simulink model "heli_q8_lab3_2020b"  (R2020b)
settings: Solver=ode1  StartTime=0.0  StopTime=inf  FixedStep=0.002  RelTol=1e-3  EnableMultiTasking=on
PostLoadFcn:
  | qc_set_target_type(getConfigSet(bdroot, 'QUARC Default Target Configuration'));
values from neighbouring files (symbols this model uses):
  A_est = [0 1 0 0 0 ... (first row only)    [init_heli_3_10_part_4.m]
  B_est = [0  0 ... (first row only)    [init_heli_3_10_part_4.m]
  C_est = eye(5)    [init_heli_3_10_part_4.m]
  elev_const = 0.53    [init_heli_3_10_part_4.m]
  F_2 = [K_2(1,1) K_2(1,3) ... (first row only)    [init_heli_3_10_part_4.m]
  gyro_bias = [0.0392850152533 -0.00867648252983 0.000660862987064]    [imu_bias.mat]    (also in update_imu_bias.m = mean(d(idx,13:15))')
  imu_bias = [-0.0918732538603 0 0.0496947738021 0 0]    [imu_bias.mat]    (also in update_imu_bias.m = imu_bias + mean(d(idx,2:6) - d(idx,8:12))')
  Joystick_gain_x = 1    [init_heli_3_10_part_4.m]
  Joystick_gain_y = -1    [init_heli_3_10_part_4.m]
  K_2 = lqr(A_lqr,B_lqr,Q_lqr, R_lqr)    [init_heli_3_10_part_4.m]
  L_est = transpose(place(transpose(A_est),transpose(C_est),p_est))    [init_heli_3_10_part_4.m]
  V_s_0 = 7.77    [init_heli_3_10_part_4.m]
undefined symbols (not defined in the file or in its folder): HIL, qc_get_step_size, sigbuilder_block
libraries: quarc_library x9
settings Model: SimulationMode=external  ExtModeTrigDuration=50000  Creator=Rchan  LastModifiedBy=saavim
settings SolverCC: PositivePriorityOrder=on
settings DataIOCC: LimitDataPoints=on  SaveFormat=Array  SignalLoggingSaveFormat=ModelDataLogs  ReturnWorkspaceOutputs=off
settings OptimizationCC: ExpressionDepthLimit=2147483647  InitFltsAndDblsToZero=on  LifeSpan=inf
settings DebuggingCC: SaveWithParameterizedLinksMsg=none  UnderspecifiedInitializationDetection=Classic  MergeDetectMultiDrivingBlocksExec=none  SolverPrmCheckMsg=warning  MultiTaskDSMMsg=warning  MultiTaskCondExecSysMsg=none  FcnCallInpInsideContextMsg=warning  AllowSymbolicDim=off  StateNameClashWarn=warning  SFUnexpectedBacktrackingDiag=warning  SFNoUnconditionalDefaultTransitionDiag=warning  SFExecutionAtInitializationDiag=none  ArithmeticOperatorsInVariantConditions=warning
settings HardwareCC: ProdBitPerPointer=32  ProdBitPerSizeT=32  ProdBitPerPtrDiffT=32  ProdLargestAtomicFloat=None  ProdIntDivRoundTo=Undefined  ProdEndianess=Unspecified  ProdWordSize=32  ProdHWDeviceType=32-bit Generic
settings ModelReferenceCC: PropagateSignalLabelsOutOfModel=off
settings SFSimCC: SimUseLocalCustomCode=off  CustomCodeUndefinedFunction=UseInterfaceOnly
settings RTWCC: Description=QUARC Win64 Target  SystemTargetFile=quarc_win64.tlc  TemplateMakefile=quarc_default_tmf  RTWUseLocalCustomCode=off
settings CodeAppCC: StateflowObjectComments=on
settings STFCustomTargetCC: MatFileLogging=on
settings GRTTargetCC: TargetLangStandard=C89/C90 (ANSI)  ParMdlRefBuildCompliant=off  CompOptLevelCompliant=off  CombineOutputUpdateFcns=off  GRTInterface=on  UseToolchainInfoCompliant=off  ExtMode=on  ExtModeMexFile=quarc_comm
settings ConfigComp: CovMetricSettings=de  CovSaveCumulativeToWorkspaceVar=on  CovSaveSingleToWorkspaceVar=on  CovExternalEMLEnable=off  CovSFcnEnable=off

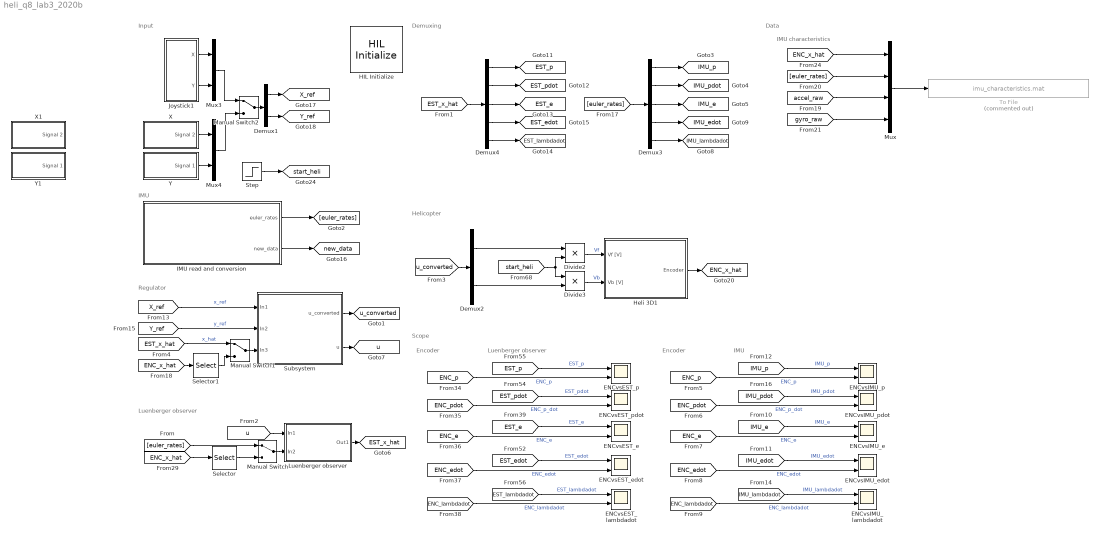
== system heli_q8_lab3_2020b ==
  note: IMU characteristics
  note: Demuxing
  note: Helicopter
  note: Luenberger observer
  note: Regulator
  note: Input
  note: IMU
  note: Scope
  note: Data
  note: Luenberger observer
  note: Encoder
  note: IMU
  note: Encoder
  Demux1 : Demux  Outputs=2
  Demux2 : Demux  Outputs=2
  Demux3 : Demux  Outputs=5
  Demux4 : Demux  Outputs=5
  Divide2 : Product  Inputs=**
  Divide3 : Product  Inputs=**
  ENCvsEST_e : Scope  NumInputPorts=2
  ENCvsEST_edot : Scope  NumInputPorts=2
  ENCvsEST_lambdadot : Scope  NumInputPorts=2
  ENCvsEST_p : Scope  NumInputPorts=2
  ENCvsEST_pdot : Scope  NumInputPorts=2
  ENCvsIMU_e : Scope  NumInputPorts=2
  ENCvsIMU_edot : Scope  NumInputPorts=2
  ENCvsIMU_lambdadot : Scope  NumInputPorts=2
  ENCvsIMU_p : Scope  NumInputPorts=2
  ENCvsIMU_pdot : Scope  NumInputPorts=2
  HIL Initialize : quarc_library/Data Acquisition/Generic/Configuration/HIL Initialize  Priority=-99  object_name=HIL-1  board_type=q8_usb  board_number=0  board_options=update_rate=normal;decimation=1  exclusive=off  active=off  hardware_clocks=[0:2]  clock_modes=[]  initial_clock_frequencies=[]  set_clock_params_at_start=off  set_clock_params_at_switch_in=off  set_clock_frequencies_at_start=off  set_clock_frequencies_at_switch_in=off  analog_input_channels=[0:7]  analog_input_configurations=[]  analog_input_maximums=10  analog_input_minimums=-10  set_analog_input_params_at_start=on  set_analog_input_params_at_switch_in=off  analog_output_channels=[0:7]  analog_output_maximums=10  analog_output_minimums=-10  initial_analog_outputs=[0]  final_analog_outputs=[0]  watchdog_analog_outputs=0  set_analog_output_params_at_start=on  set_analog_output_params_at_switch_in=off  set_analog_outputs_at_start=on  set_analog_outputs_at_switch_in=off  set_analog_outputs_at_terminate=on  set_analog_outputs_at_switch_out=off  set_analog_outputs_on_watchdog=off  digital_input_channels=[]  digital_output_channels=[]  digital_output_configuration=[]  initial_digital_outputs=[1]  final_digital_outputs=[1]  watchdog_digital_outputs=[1]  set_digital_output_params_at_start=off  set_digital_output_params_at_switch_in=off  set_digital_outputs_at_start=on  set_digital_outputs_at_switch_in=off  set_digital_outputs_at_terminate=on  set_digital_outputs_at_switch_out=off  set_digital_outputs_on_watchdog=off  encoder_channels=[0:7]  quadrature=[4]  encoder_filter_frequency=[]  initial_encoder_counts=[0]  set_encoder_params_at_start=on  set_encoder_params_at_switch_in=off  set_encoder_counts_at_start=on  set_encoder_counts_at_switch_in=off  pwm_channels=[0:7]  pwm_modes=0  pwm_frequency=99.532799999999995e6/4095  pwm_configuration=[0]  pwm_alignment=[0]  pwm_polarity=[1]  pwm_leading_deadband=[0]  pwm_trailing_deadband=[0]  initial_pwm_outputs=[0]  final_pwm_outputs=[0]  watchdog_pwm_outputs=[0]  set_pwm_params_at_start=on  set_pwm_params_at_switch_in=off  set_pwm_outputs_at_start=on  set_pwm_outputs_at_switch_in=off  set_pwm_outputs_at_terminate=on  set_pwm_outputs_at_switch_out=off  set_pwm_outputs_on_watchdog=off  other_output_channels=[]  initial_other_outputs=[]  final_other_outputs=[]  watchdog_other_outputs=[]  set_other_outputs_at_start=off  set_other_outputs_at_switch_in=off  set_other_outputs_at_terminate=off  set_other_outputs_at_switch_out=off  set_other_outputs_on_watchdog=off
  Heli 3D1 : Subsystem
  IMU read and conversion : Subsystem
  Joystick1 : Subsystem
  Luenberger observer : Subsystem
  Manual Switch : ManualSwitch
  Manual Switch1 : ManualSwitch
  Manual Switch2 : ManualSwitch
  Mux : Mux
  Mux3 : Mux  Inputs=2
  Mux4 : Mux  Inputs=2
  Selector : Selector  InputPortWidth=6  IndexOptions=Index vector (dialog)  Indices=[1 2 3 4 6]  OutputSizes=1
  Selector1 : Selector  InputPortWidth=6  IndexOptions=Index vector (dialog)  Indices=[1 2 3 4 6]  OutputSizes=1
  Step : Step  Time=3  SampleTime=0
  Subsystem : Subsystem
  To File : ToFile  Commented=on  Filename=imu_characteristics.mat  MatrixName=imu_characteristics  SampleTime=0.002
  X : Subsystem  Tag=STV Subsys  LoadFcn=sigbuilder_block('load');  StartFcn=sigbuilder_block('start');  StopFcn=sigbuilder_block('stop');  ClipboardFcn=sigbuilder_block('clipboard');  mask(Sigbuilder block){tuvar=[0:10]}
      mask help: Simulink:masks:SigbuilderBlock_MD
      mask init:
      | if ~strcmp(get_param(bdroot(gcbh),'SimulationStatus'),'stopped') tuvar = sigbuilder_block('maskInit'); end
      settings: CopyFcn=sigbuilder_block('copy');  DeleteFcn=sigbuilder_block('delete');  ModelCloseFcn=sigbuilder_block('modelClose');  PreSaveFcn=sigbuilder_block('preSave');  PauseFcn=sigbuilder_block('pause');  ContinueFcn=sigbuilder_block('continue');  NameChangeFcn=sigbuilder_block('namechange');  OpenFcn=sigbuilder_block('open',[0 172 1440 619 ]);  CloseFcn=sigbuilder_block('close');
      mask Display: plot(0, 0, 100, 100,[2, 2, 32, 32, 2], [68, 8, 8, 68, 68],[32, 2], [38, 38], [32, 19, 2],[53, 60, 44], [32, 17, 17, 2],[16, 16, 31, 31]);txt = getActiveGroup(gcbh);text(2, 100, txt,'verticalAlignment', 'top');
  X1 : Subsystem  Tag=STV Subsys  LoadFcn=sigbuilder_block('load');  StartFcn=sigbuilder_block('start');  StopFcn=sigbuilder_block('stop');  ClipboardFcn=sigbuilder_block('clipboard');  mask(Sigbuilder block){tuvar=[0:10]}
      mask help: Simulink:masks:SigbuilderBlock_MD
      mask init:
      | if ~strcmp(get_param(bdroot(gcbh),'SimulationStatus'),'stopped') tuvar = sigbuilder_block('maskInit'); end
      settings: CopyFcn=sigbuilder_block('copy');  DeleteFcn=sigbuilder_block('delete');  ModelCloseFcn=sigbuilder_block('modelClose');  PreSaveFcn=sigbuilder_block('preSave');  PauseFcn=sigbuilder_block('pause');  ContinueFcn=sigbuilder_block('continue');  NameChangeFcn=sigbuilder_block('namechange');  OpenFcn=sigbuilder_block('open',[0 172 1440 619 ]);  CloseFcn=sigbuilder_block('close');
      mask Display: plot(0, 0, 100, 100,[2, 2, 32, 32, 2], [68, 8, 8, 68, 68],[32, 2], [38, 38], [32, 19, 2],[53, 60, 44], [32, 17, 17, 2],[16, 16, 31, 31]);txt = getActiveGroup(gcbh);text(2, 100, txt,'verticalAlignment', 'top');
  Y : Subsystem  Tag=STV Subsys  LoadFcn=sigbuilder_block('load');  StartFcn=sigbuilder_block('start');  StopFcn=sigbuilder_block('stop');  ClipboardFcn=sigbuilder_block('clipboard');  mask(Sigbuilder block){tuvar=[0:10]}
      mask help: Simulink:masks:SigbuilderBlock_MD
      mask init:
      | if ~strcmp(get_param(bdroot(gcbh),'SimulationStatus'),'stopped') tuvar = sigbuilder_block('maskInit'); end
      settings: CopyFcn=sigbuilder_block('copy');  DeleteFcn=sigbuilder_block('delete');  ModelCloseFcn=sigbuilder_block('modelClose');  PreSaveFcn=sigbuilder_block('preSave');  PauseFcn=sigbuilder_block('pause');  ContinueFcn=sigbuilder_block('continue');  NameChangeFcn=sigbuilder_block('namechange');  OpenFcn=sigbuilder_block('open',[217.5 306 1336.5 574.5 ]);  CloseFcn=sigbuilder_block('close');
      mask Display: plot(0, 0, 100, 100,[2, 2, 32, 32, 2], [68, 8, 8, 68, 68],[32, 2], [38, 38], [32, 19, 2],[53, 60, 44], [32, 17, 17, 2],[16, 16, 31, 31]);txt = getActiveGroup(gcbh);text(2, 100, txt,'verticalAlignment', 'top');
  Y1 : Subsystem  Tag=STV Subsys  LoadFcn=sigbuilder_block('load');  StartFcn=sigbuilder_block('start');  StopFcn=sigbuilder_block('stop');  ClipboardFcn=sigbuilder_block('clipboard');  mask(Sigbuilder block){tuvar=[0:10]}
      mask help: Simulink:masks:SigbuilderBlock_MD
      mask init:
      | if ~strcmp(get_param(bdroot(gcbh),'SimulationStatus'),'stopped') tuvar = sigbuilder_block('maskInit'); end
      settings: CopyFcn=sigbuilder_block('copy');  DeleteFcn=sigbuilder_block('delete');  ModelCloseFcn=sigbuilder_block('modelClose');  PreSaveFcn=sigbuilder_block('preSave');  PauseFcn=sigbuilder_block('pause');  ContinueFcn=sigbuilder_block('continue');  NameChangeFcn=sigbuilder_block('namechange');  OpenFcn=sigbuilder_block('open',[217.5 306 1336.5 574.5 ]);  CloseFcn=sigbuilder_block('close');
      mask Display: plot(0, 0, 100, 100,[2, 2, 32, 32, 2], [68, 8, 8, 68, 68],[32, 2], [38, 38], [32, 19, 2],[53, 60, 44], [32, 17, 17, 2],[16, 16, 31, 31]);txt = getActiveGroup(gcbh);text(2, 100, txt,'verticalAlignment', 'top');
  tag scope: ENC_x_hat=global, EST_e=global, EST_edot=global, EST_lambdadot=global, EST_p=global, EST_pdot=global, EST_x_hat=global, IMU_e=global, IMU_edot=global, IMU_lambdadot=global, IMU_p=global, IMU_pdot=global, X_ref=global, Y_ref=global, new_data=global, start_heli=global, u=global, u_converted=global
  wires:
  Demux4/1 -> [EST_p]
  Demux4/2 -> [EST_pdot]
  Demux4/3 -> [EST_e]
  Demux4/4 -> [EST_edot]
  Demux4/5 -> [EST_lambdadot]
  X/1(Signal 2) -> Mux4/1
  Manual Switch2/1 -> Demux1/1
  Y/1(Signal 1) -> Mux4/2
  Demux1/1 -> [X_ref]
  Joystick1/1(X) -> Mux3/1
  Mux3/1 -> Manual Switch2/1
  Demux1/2 -> [Y_ref]
  Joystick1/2(Y) -> Mux3/2
  Step/1 -> [start_heli]
  Mux4/1 -> Manual Switch2/2
  [EST_x_hat] -> Demux4/1
  [X_ref] -> Subsystem/1(In1)  "x_ref"
  [Y_ref] -> Subsystem/2(In2)  "y_ref"
  Subsystem/1(u_converted) -> [u_converted]
  Subsystem/2(u) -> [u]
  Manual Switch/1 -> Luenberger observer/2(In2)
  [u] -> Luenberger observer/1(In1)
  [euler_rates] -> Manual Switch/1
  Luenberger observer/1(Out1) -> [EST_x_hat]
  Demux2/1 -> Divide2/1
  Demux2/2 -> Divide3/2
  [u_converted] -> Demux2/1
  [start_heli] -> Divide3/1, Divide2/2
  Heli 3D1/1(Encoder) -> [ENC_x_hat]
  IMU read and conversion/1(euler_rates) -> [euler_rates]
  IMU read and conversion/2(new_data) -> [new_data]
  [ENC_x_hat] -> Selector/1
  Selector/1 -> Manual Switch/2
  [ENC_edot] -> ENCvsEST_edot/2  "ENC_edot"
  [ENC_lambdadot] -> ENCvsEST_lambdadot/2  "ENC_lambdadot"
  [EST_lambdadot] -> ENCvsEST_lambdadot/1  "EST_lambdadot"
  [EST_edot] -> ENCvsEST_edot/1  "EST_edot"
  [EST_p] -> ENCvsEST_p/1  "EST_p"
  [IMU_pdot] -> ENCvsIMU_pdot/1  "IMU_pdot"
  [ENC_pdot] -> ENCvsEST_pdot/2  "ENC_p_dot"
  [EST_e] -> ENCvsEST_e/1  "EST_e"
  [IMU_p] -> ENCvsIMU_p/1  "IMU_p"
  [ENC_p] -> ENCvsEST_p/2  "ENC_p"
  [ENC_edot] -> ENCvsIMU_edot/2  "ENC_edot"
  [IMU_edot] -> ENCvsIMU_edot/1  "IMU_edot"
  [ENC_lambdadot] -> ENCvsIMU_lambdadot/2  "ENC_lambdadot"
  [ENC_e] -> ENCvsEST_e/2  "ENC_e"
  [IMU_lambdadot] -> ENCvsIMU_lambdadot/1  "IMU_lambdadot"
  [EST_pdot] -> ENCvsEST_pdot/1  "EST_pdot"
  [ENC_e] -> ENCvsIMU_e/2  "ENC_e"
  [ENC_pdot] -> ENCvsIMU_pdot/2  "ENC_p_dot"
  [IMU_e] -> ENCvsIMU_e/1  "IMU_e"
  [ENC_p] -> ENCvsIMU_p/2  "ENC_p"
  [euler_rates] -> Demux3/1
  Demux3/3 -> [IMU_e]
  Demux3/4 -> [IMU_edot]
  Demux3/5 -> [IMU_lambdadot]
  Demux3/2 -> [IMU_pdot]
  Demux3/1 -> [IMU_p]
  [EST_x_hat] -> Manual Switch1/1  "x_hat"
  Manual Switch1/1 -> Subsystem/3(In3)
  Selector1/1 -> Manual Switch1/2
  [ENC_x_hat] -> Selector1/1
  [ENC_x_hat] -> Mux/1
  [euler_rates] -> Mux/2
  [accel_raw] -> Mux/3
  [gyro_raw] -> Mux/4
  Mux/1 -> To File/1
  Divide2/1 -> Heli 3D1/1(Vf [V])  "Vf"
  Divide3/1 -> Heli 3D1/2(Vb [V])  "Vb"

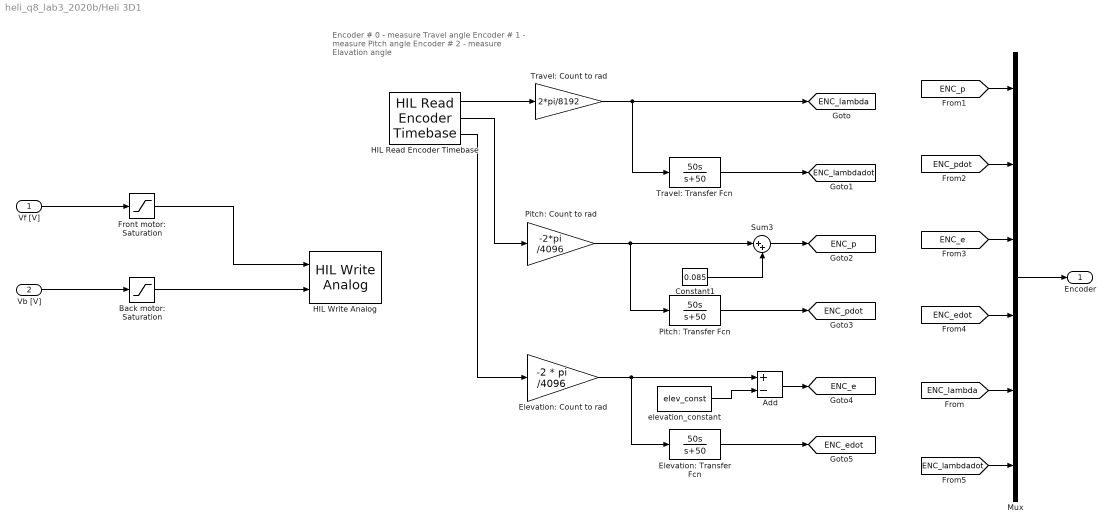
== system heli_q8_lab3_2020b/Heli 3D1 ==
  note: Encoder # 0 - measure Travel angle
      | Encoder # 1 - measure Pitch angle
      | Encoder # 2 - measure Elavation angle
  Vf [V] : Inport
  Vb [V] : Inport  Port=2
  Add : Sum  Inputs=+-
  Back motor: Saturation : Saturate  UpperLimit=5  LowerLimit=-5
  Constant1 : Constant  Value=0.085
  Elevation: Count to rad : Gain  Gain=-2 * pi /4096
  Elevation: Transfer Fcn : TransferFcn  Numerator=[50 0]  Denominator=[1 50]
  Front motor: Saturation : Saturate  UpperLimit=5  LowerLimit=-5
  HIL Read Encoder Timebase : quarc_library/Data Acquisition/Generic/Timebases/HIL Read Encoder Timebase  object_name=HIL-1  clock=0  channels=[0:2]  active=on  vector_output=off  data_type_mode=Inherit via back propagation  data_type=double  overflow_mode=Error on overflow  samples_in_buffer=max(ceil(1/qc_get_step_size), 1)
  HIL Write Analog : quarc_library/Data Acquisition/Generic/Immediate I//O/HIL Write Analog  object_name=HIL-1  channels=[0:1]  sample_time=-1  active=off  vector_input=off
  Mux : Mux  Inputs=6
  Pitch: Count to rad : Gain  Gain=-2*pi /4096
  Pitch: Transfer Fcn : TransferFcn  Numerator=[50 0]  Denominator=[1 50]
  Sum3 : Sum  Inputs=|++
  Travel: Count to rad : Gain  Gain=2*pi/8192
  Travel: Transfer Fcn : TransferFcn  Numerator=[50 0]  Denominator=[1 50]
  elevation_constant : Constant  Value=elev_const
  Encoder : Outport
  tag scope: ENC_e=global, ENC_edot=global, ENC_lambda=global, ENC_lambdadot=global, ENC_p=global, ENC_pdot=global
  wires:
  HIL Read Encoder Timebase/1 -> Travel: Count to rad/1
  HIL Read Encoder Timebase/2 -> Pitch: Count to rad/1
  HIL Read Encoder Timebase/3 -> Elevation: Count to rad/1
  Travel: Count to rad/1 -> Travel: Transfer Fcn/1, [ENC_lambda]
  Travel: Transfer Fcn/1 -> [ENC_lambdadot]
  Elevation: Count to rad/1 -> Add/1, Elevation: Transfer Fcn/1
  Elevation: Transfer Fcn/1 -> [ENC_edot]
  Vf [V]/1 -> Front motor: Saturation/1
  Vb [V]/1 -> Back motor: Saturation/1
  Front motor: Saturation/1 -> HIL Write Analog/1
  Back motor: Saturation/1 -> HIL Write Analog/2
  elevation_constant/1 -> Add/2
  Add/1 -> [ENC_e]
  Pitch: Count to rad/1 -> Pitch: Transfer Fcn/1, Sum3/1
  Pitch: Transfer Fcn/1 -> [ENC_pdot]
  Constant1/1 -> Sum3/2
  Sum3/1 -> [ENC_p]
  Mux/1 -> Encoder/1
  [ENC_p] -> Mux/1
  [ENC_pdot] -> Mux/2
  [ENC_lambdadot] -> Mux/6
  [ENC_lambda] -> Mux/5
  [ENC_edot] -> Mux/4
  [ENC_e] -> Mux/3

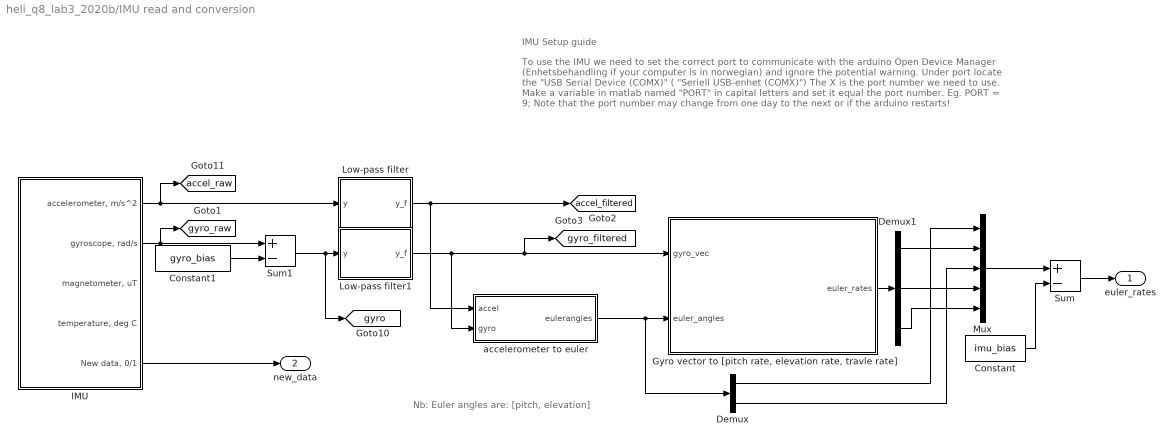
== system heli_q8_lab3_2020b/IMU read and conversion ==
  note: Nb: Euler angles are: [pitch, elevation]
  note: IMU Setup guide
  note: To use the IMU we need to set the correct port to communicate with the arduino
      | Open Device Manager (Enhetsbehandling if your computer is in norwegian) and ignore the potential warning.
      | Under port locate the "USB Serial Device (COMX)" ( "Seriell USB-enhet (COMX)")
      | The X is the port number we need to use.
      |
      | Make a variable in matlab named "PORT" in capital letters and set it equal the port number.
      | Eg.
      | PORT = 9;
      |
      | Note that the port number may change from one day to the next or if the arduino restarts!
  Constant : Constant  Value=imu_bias
  Constant1 : Constant  Value=gyro_bias
  Demux : Demux  Outputs=2
  Demux1 : Demux  Outputs=3
  "Gyro vector to [pitch rate, elevation rate, travle rate]" : MATLAB Function  TreatAsAtomicUnit=on
  IMU : Subsystem
  Low-pass filter : MATLAB Function  TreatAsAtomicUnit=on
  Low-pass filter1 : MATLAB Function  TreatAsAtomicUnit=on
  Mux : Mux  Inputs=5
  Sum : Sum  Inputs=+-
  Sum1 : Sum  Inputs=+-
  accelerometer to euler : MATLAB Function  TreatAsAtomicUnit=on
  euler_rates : Outport
  new_data : Outport  Port=2
  tag scope: accel_filtered=global, accel_raw=global, gyro=global, gyro_filtered=global, gyro_raw=global
  wires:
  IMU/2("gyroscope, rad/s") -> Sum1/1, [gyro_raw]
  "Gyro vector to [pitch rate, elevation rate, travle rate]"/1(euler_rates) -> Demux1/1
  Demux/1 -> Mux/1
  Demux1/1 -> Mux/2
  Demux/2 -> Mux/3
  Demux1/2 -> Mux/4
  Demux1/3 -> Mux/5
  IMU/5("New data, 0/1") -> new_data/1
  IMU/1("accelerometer, m/s^2") -> [accel_raw], Low-pass filter/1(y)
  accelerometer to euler/1(eulerangles) -> Demux/1, "Gyro vector to [pitch rate, elevation rate, travle rate]"/2(euler_angles)
  Constant/1 -> Sum/2
  Constant1/1 -> Sum1/2
  Sum1/1 -> [gyro], Low-pass filter1/1(y)
  Sum/1 -> euler_rates/1
  Mux/1 -> Sum/1
  Low-pass filter/1(y_f) -> [accel_filtered], accelerometer to euler/1(accel)
  Low-pass filter1/1(y_f) -> [gyro_filtered], "Gyro vector to [pitch rate, elevation rate, travle rate]"/1(gyro_vec), accelerometer to euler/2(gyro)

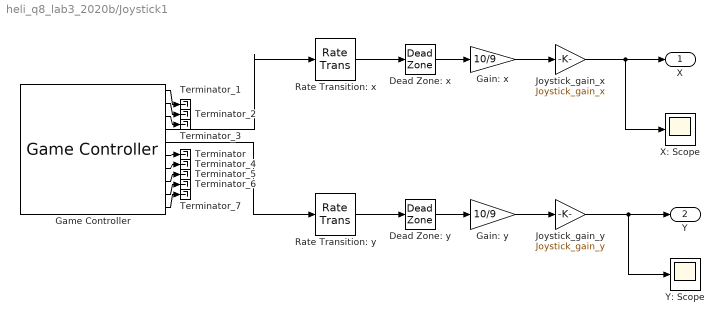
== system heli_q8_lab3_2020b/Joystick1 ==
  Dead Zone: x : DeadZone  LowerValue=-0.1  UpperValue=0.1  SaturateOnIntegerOverflow=on
  Dead Zone: y : DeadZone  LowerValue=-0.1  UpperValue=0.1  SaturateOnIntegerOverflow=on
  Gain: x : Gain  Gain=10/9
  Gain: y : Gain  Gain=10/9
  Game Controller : quarc_library/Devices/Peripherals/Target/Game Controller  controller=1  buffer_size=12  deadzone=[]  saturation=[]  sample_time=max(qc_get_step_size, 0.01)  auto_center=off  enabled=on
      settings: SourceProductName=QUARC Targets
  Joystick_gain_x : Gain  Gain=Joystick_gain_x
  Joystick_gain_y : Gain  Gain=Joystick_gain_y
  Rate Transition: x : RateTransition
  Rate Transition: y : RateTransition
  Terminator : Terminator
  Terminator_{1..7} (7 alike) : Terminator
  X: Scope : Scope
  Y: Scope : Scope
  X : Outport
  Y : Outport  Port=2
  wires:
  Rate Transition: y/1 -> Dead Zone: y/1
  Rate Transition: x/1 -> Dead Zone: x/1
  Game Controller/5 -> Rate Transition: y/1
  Game Controller/4 -> Rate Transition: x/1
  Game Controller/1 -> Terminator_1/1
  Game Controller/2 -> Terminator_2/1
  Game Controller/7 -> Terminator_4/1
  Game Controller/8 -> Terminator_5/1
  Game Controller/9 -> Terminator_6/1
  Game Controller/10 -> Terminator_7/1
  Game Controller/6 -> Terminator/1
  Dead Zone: x/1 -> Gain: x/1
  Dead Zone: y/1 -> Gain: y/1
  Gain: x/1 -> Joystick_gain_x/1
  Gain: y/1 -> Joystick_gain_y/1
  Joystick_gain_x/1 -> X/1, X: Scope/1
  Joystick_gain_y/1 -> Y: Scope/1, Y/1
  Game Controller/3 -> Terminator_3/1

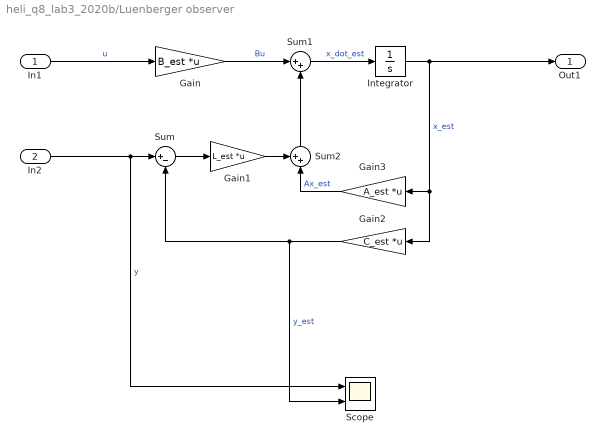
== system heli_q8_lab3_2020b/Luenberger observer ==
  In1 : Inport
  In2 : Inport  Port=2
  Gain : Gain  Gain=B_est  Multiplication=Matrix(K*u)
  Gain1 : Gain  Gain=L_est  Multiplication=Matrix(K*u)
  Gain2 : Gain  Gain=C_est  Multiplication=Matrix(K*u)
  Gain3 : Gain  Gain=A_est  Multiplication=Matrix(K*u)
  Integrator : Integrator
  Scope : Scope  NumInputPorts=2
  Sum : Sum  Inputs=|+-
  Sum1 : Sum  Inputs=|++
  Sum2 : Sum  Inputs=++|
  Out1 : Outport
  wires:
  In1/1 -> Gain/1  "u"
  In2/1 -> Scope/1, Sum/1  "y"
  Gain/1 -> Sum1/1  "Bu"
  Sum/1 -> Gain1/1
  Sum1/1 -> Integrator/1  "x_dot_est"
  Integrator/1 -> Gain2/1, Gain3/1, Out1/1  "x_est"
  Gain2/1 -> Scope/2, Sum/2  "y_est"
  Gain1/1 -> Sum2/1
  Sum2/1 -> Sum1/2
  Gain3/1 -> Sum2/2  "Ax_est"

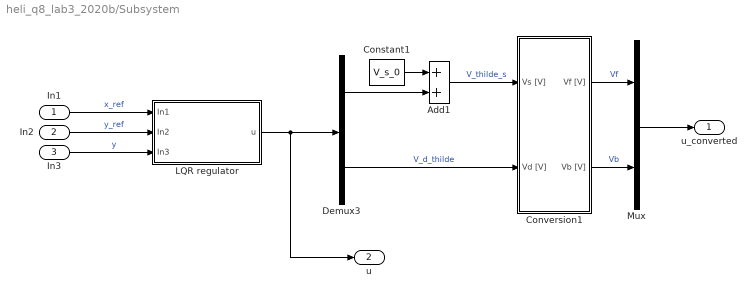
== system heli_q8_lab3_2020b/Subsystem ==
  In1 : Inport
  In2 : Inport  Port=2
  In3 : Inport  Port=3
  Add1 : Sum
  Constant1 : Constant  Value=V_s_0
  Conversion1 : Subsystem
  Demux3 : Demux  Outputs=2
  LQR regulator : Subsystem
  Mux : Mux  Inputs=2
  u_converted : Outport
  u : Outport  Port=2
  wires:
  Add1/1 -> Conversion1/1(Vs [V])  "V_thilde_s"
  Demux3/2 -> Conversion1/2(Vd [V])  "V_d_thilde"
  Conversion1/2(Vb [V]) -> Mux/2  "Vb"
  Constant1/1 -> Add1/1
  In1/1 -> LQR regulator/1(In1)  "x_ref"
  In3/1 -> LQR regulator/3(In3)  "y"
  Mux/1 -> u_converted/1
  LQR regulator/1(u) -> u/1, Demux3/1
  Conversion1/1(Vf [V]) -> Mux/1  "Vf"
  In2/1 -> LQR regulator/2(In2)  "y_ref"
  Demux3/1 -> Add1/2

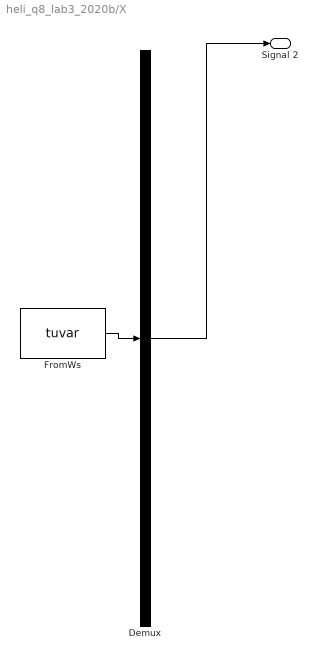
== system heli_q8_lab3_2020b/X ==
  Demux : Demux  Tag=STV Demux  Outputs=1
      settings: DisplayOption=none
  FromWs : FromWorkspace  Tag=STV FromWs  VariableName=tuvar
      SigBuilderData=|
      | common.afterFinalStr = 'Extrapolate'
      | common.sampleTime = 0
      | dataSet.timeRange = [0 90]
      | dataSet.name = 'Group 1'
      | sbobj.Groups.Name = 'Group 1'
      | sbobj.Groups.Signals.Name = 'Signal 2'
      | sbobj.Groups.Signals.XData = [0 35 35 40 40 45 45 50 50 55 55 65 65 70 70 80 80 90]
      | sbobj.Groups.Signals.YData = [0 0 0.25 0.25 0 0 -0.25 -0.25 0 0 0.099 0.099 0 0 -0.131 -0.131 0 0]
      | sbobj.Groups.TimeRange = [0 90]
  Signal 2 : Outport  Tag=STV Outport
  wires:
  Demux/1 -> Signal 2/1
  FromWs/1 -> Demux/1

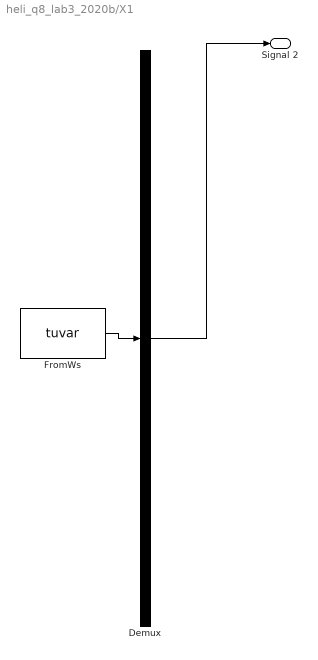
== system heli_q8_lab3_2020b/X1 ==
  Demux : Demux  Tag=STV Demux  Outputs=1
      settings: DisplayOption=none
  FromWs : FromWorkspace  Tag=STV FromWs  VariableName=tuvar
      SigBuilderData=|
      | common.afterFinalStr = 'Extrapolate'
      | common.sampleTime = 0
      | dataSet.timeRange = [0 60]
      | dataSet.name = 'Group 1'
      | sbobj.Groups.Name = 'Group 1'
      | sbobj.Groups.Signals.Name = 'Signal 2'
      | sbobj.Groups.Signals.XData = [0 10 10 15 15 30 30 35 35 60]
      | sbobj.Groups.Signals.YData = [0 0 0.4 0.4 0 0 -0.4 -0.4 0 0]
      | sbobj.Groups.TimeRange = [0 60]
  Signal 2 : Outport  Tag=STV Outport
  wires:
  Demux/1 -> Signal 2/1
  FromWs/1 -> Demux/1

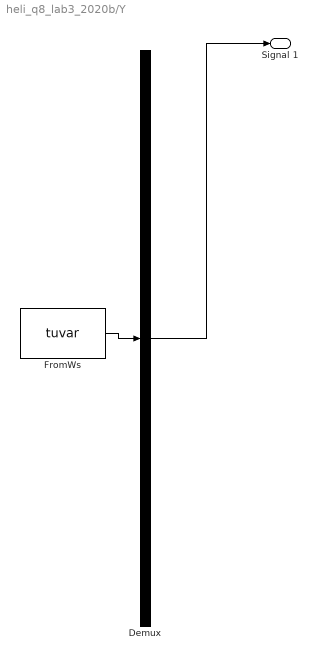
== system heli_q8_lab3_2020b/Y ==
  Demux : Demux  Tag=STV Demux  Outputs=1
      settings: DisplayOption=none
  FromWs : FromWorkspace  Tag=STV FromWs  VariableName=tuvar
      SigBuilderData=|
      | common.afterFinalStr = 'Extrapolate'
      | common.sampleTime = 0
      | dataSet.timeRange = [0 90]
      | dataSet.name = 'Group 1'
      | sbobj.Groups.Name = 'Group 1'
      | sbobj.Groups.Signals.Name = 'Signal 1'
      | sbobj.Groups.Signals.XData = [0 4 4 10 10 20 20 23 23 27 27 30 30 90]
      | sbobj.Groups.Signals.YData = [0 0 0.101 0.101 0 0 -0.2 -0.2 0 0 0.2 0.2 0 0]
      | sbobj.Groups.TimeRange = [0 90]
  Signal 1 : Outport  Tag=STV Outport
  wires:
  Demux/1 -> Signal 1/1
  FromWs/1 -> Demux/1

== system heli_q8_lab3_2020b/Y1 ==
  Demux : Demux  Tag=STV Demux  Outputs=1
      settings: DisplayOption=none
  FromWs : FromWorkspace  Tag=STV FromWs  VariableName=tuvar
      SigBuilderData=|
      | common.afterFinalStr = 'Extrapolate'
      | common.sampleTime = 0
      | dataSet.timeRange = [0 10]
      | dataSet.name = 'Group 1'
      | sbobj.Groups.Name = 'Group 1'
      | sbobj.Groups.Signals.Name = 'Signal 1'
      | sbobj.Groups.Signals.XData = [0 5.01 5.01 6 6 10]
      | sbobj.Groups.Signals.YData = [0 0 0.4 0.4 0 0]
  Signal 1 : Outport  Tag=STV Outport
  wires:
  Demux/1 -> Signal 1/1
  FromWs/1 -> Demux/1

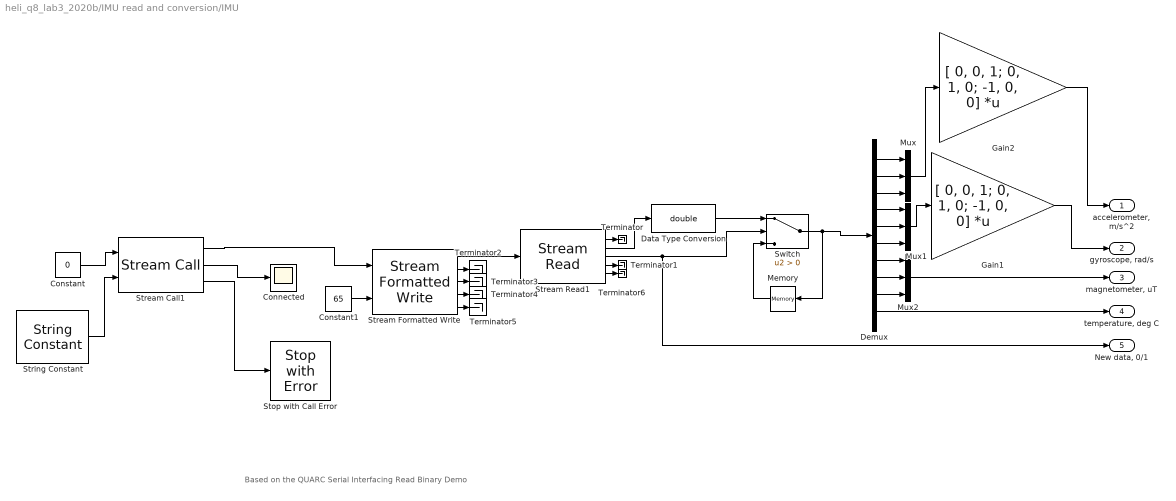
== system heli_q8_lab3_2020b/IMU read and conversion/IMU ==
  note: Based on the QUARC Serial Interfacing Read Binary Demo
  Connected : Scope
  Constant : Constant  Value=0
  Constant1 : Constant  Value=65
  Data Type Conversion : DataTypeConversion  OutDataTypeStr=double
  Demux : Demux  Outputs=10
  Gain1 : Gain  Gain=[ 0, 0, 1; 0, 1, 0; -1, 0, 0]  Multiplication=Matrix(K*u) (u vector)
  Gain2 : Gain  Gain=[ 0, 0, 1; 0, 1, 0; -1, 0, 0]  Multiplication=Matrix(K*u) (u vector)
  Memory : Memory  InitialCondition=[0 0 0 0 0 0 0 0 0 0]
  Mux : Mux  Inputs=3
  Mux1 : Mux  Inputs=3
  Mux2 : Mux  Inputs=3
  Stop with Call Error : quarc_library/Sinks/Error Handling/Stop with Error  message_type=Interpret input as error code  message=Error occurred
      settings: SourceProductName=QUARC Targets
  Stream Call1 : quarc_library/Communications/Intermediate/Stream Call  uri_source=External input port  uri=serial://IMU:9?baud=115200,word=8,parity=none,stop=1,flow='none'  apply_uri_to_all_configs=on  send_buffer_size=8000  receive_buffer_size=8000  byte_order=little endian (Intel - LSB first)  sample_time=qc_get_step_size  non_blocking=on  active=off
      settings: SourceProductName=QUARC Targets
  Stream Formatted Write : quarc_library/Communications/Intermediate/Stream Formatted Write  format_string=%c\n  max_code_units=80  optimization=Minimizing latency
      settings: SourceProductName=QUARC Targets
  Stream Read1 : quarc_library/Communications/Intermediate/Stream Read  data_type=single  type_expr=BusObject  num_elements=10  receive_dims=off
      settings: SourceProductName=QUARC Targets
  String Constant : quarc_library/Strings/String Constant  string_value=qc_perform_substitutions('serial://IMU:%{PORT}?baud=115200,word=8,parity=none,stop=1')  evaluate_string=on  string_type=URI  max_length=255  sample_time=inf  variable_size=off
      settings: AttributesFormatString="\"serial://IMU:6?baud=115200,word=8,parity=none,stop=1\""  SourceProductName=QUARC Targets
  Switch : Switch  Criteria=u2 > Threshold
  Terminator{,1..6} (7 alike) : Terminator
  "accelerometer, m/s^2" : Outport
  "gyroscope, rad/s" : Outport  Port=2
  "magnetometer, uT" : Outport  Port=3
  "temperature, deg C" : Outport  Port=4
  "New data, 0/1" : Outport  Port=5
  wires:
  Switch/1 -> Memory/1, Demux/1
  Data Type Conversion/1 -> Switch/1
  Stream Read1/3 -> "New data, 0/1"/1, Switch/2
  Stream Formatted Write/1 -> Stream Read1/1
  Constant1/1 -> Stream Formatted Write/2
  Gain1/1 -> "gyroscope, rad/s"/1
  Gain2/1 -> "accelerometer, m/s^2"/1
  Stream Read1/4 -> Terminator1/1
  Demux/10 -> "temperature, deg C"/1
  Mux1/1 -> Gain1/1
  Stream Read1/2 -> Data Type Conversion/1
  Demux/7 -> Mux2/1
  Demux/8 -> Mux2/2
  Demux/9 -> Mux2/3
  Mux2/1 -> "magnetometer, uT"/1
  Demux/6 -> Mux1/3
  Demux/5 -> Mux1/2
  Demux/4 -> Mux1/1
  Mux/1 -> Gain2/1
  Demux/3 -> Mux/3
  Demux/1 -> Mux/1
  Demux/2 -> Mux/2
  Stream Read1/1 -> Terminator/1
  Stream Call1/1 -> Stream Formatted Write/1
  Constant/1 -> Stream Call1/1
  String Constant/1 -> Stream Call1/2
  Stream Call1/2 -> Connected/1
  Stream Call1/3 -> Stop with Call Error/1
  Memory/1 -> Switch/3
  Stream Formatted Write/2 -> Terminator2/1
  Stream Formatted Write/3 -> Terminator3/1
  Stream Formatted Write/4 -> Terminator4/1
  Stream Formatted Write/5 -> Terminator5/1
  Stream Read1/5 -> Terminator6/1

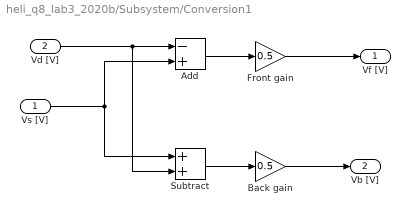
== system heli_q8_lab3_2020b/Subsystem/Conversion1 ==
  Vs [V] : Inport
  Vd [V] : Inport  Port=2
  Add : Sum  Inputs=-+
  Back gain : Gain  Gain=0.5
  Front gain : Gain  Gain=0.5
  Subtract : Sum
  Vf [V] : Outport
  Vb [V] : Outport  Port=2
  wires:
  Vd [V]/1 -> Subtract/2, Add/1
  Vs [V]/1 -> Subtract/1, Add/2
  Subtract/1 -> Back gain/1
  Back gain/1 -> Vb [V]/1
  Add/1 -> Front gain/1
  Front gain/1 -> Vf [V]/1

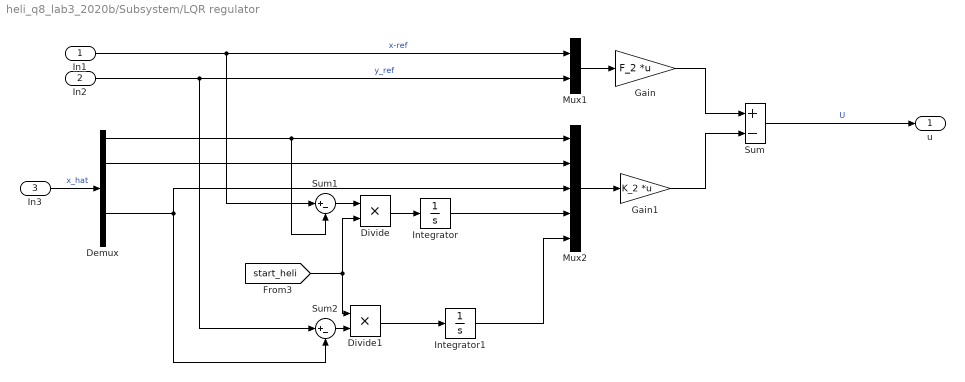
== system heli_q8_lab3_2020b/Subsystem/LQR regulator ==
  In1 : Inport
  In2 : Inport  Port=2
  In3 : Inport  Port=3
  Demux : Demux  Outputs=5
  Divide : Product  Inputs=**
  Divide1 : Product  Inputs=**
  Gain : Gain  Gain=F_2  Multiplication=Matrix(K*u)
  Gain1 : Gain  Gain=K_2  Multiplication=Matrix(K*u)
  Integrator : Integrator
  Integrator1 : Integrator
  Mux1 : Mux  Inputs=2
  Mux2 : Mux  Inputs=5
  Sum : Sum  Inputs=+-
  Sum1 : Sum  Inputs=|+-
  Sum2 : Sum  Inputs=|+-
  u : Outport
  wires:
  Demux/1 -> Sum1/2, Mux2/1
  Integrator1/1 -> Mux2/5
  Demux/2 -> Mux2/2
  Gain1/1 -> Sum/2
  Mux1/1 -> Gain/1
  Sum/1 -> u/1  "U"
  Mux2/1 -> Gain1/1
  Demux/4 -> Sum2/2, Mux2/3
  Gain/1 -> Sum/1
  Integrator/1 -> Mux2/4
  In1/1 -> Mux1/1, Sum1/1  "x-ref"
  In2/1 -> Mux1/2, Sum2/1  "y_ref"
  Sum1/1 -> Divide/1
  Divide/1 -> Integrator/1
  [start_heli] -> Divide1/1, Divide/2
  Divide1/1 -> Integrator1/1
  Sum2/1 -> Divide1/2
  In3/1 -> Demux/1  "x_hat"

== matlab function heli_q8_lab3_2020b/IMU read and conversion/Gyro vector to [pitch rate, elevation rate, travle rate] ==
  data: gyro_vec input; euler_rates output; euler_angles input
function euler_rates = gyro_vec_to_euler_rates(gyro_vec,euler_angles)
%#codegen
    phi = euler_angles(1);
    theta = euler_angles(2);
    %psi = euler_angles(3);


    T = [1, sin(phi)*tan(theta), cos(phi)*tan(theta);
         0, cos(phi),            -sin(phi);
         0, sin(phi)/cos(theta), cos(phi)/cos(theta)]; 
euler_rates = T*gyro_vec;

== matlab function heli_q8_lab3_2020b/IMU read and conversion/Low-pass filter ==
  data: y input; y_f output; fc_acc parameter
function y_f = lowpass(y, fc_acc)

persistent state
Ts = 0.002;
if isempty(state), state = y(:); end
a = exp(-2*pi*fc_acc(:)*Ts);
state = a.*state + (1 - a).*y(:);
y_f = state;
end

== matlab function heli_q8_lab3_2020b/IMU read and conversion/Low-pass filter1 ==
  data: y input; y_f output; fc_gyro parameter
function y_f = lowpass(y, fc_gyro)

persistent state
Ts = 0.002;
if isempty(state), state = y(:); end
a = exp(-2*pi*fc_gyro(:)*Ts);
state = a.*state + (1 - a).*y(:);
y_f = state;
end

== matlab function heli_q8_lab3_2020b/IMU read and conversion/accelerometer to euler ==
  data: accel input; eulerangles output; gyro input
function eulerangles = fcn(accel, gyro)
l_h = 0.66; %Avstand elevasjonsakse - hode [m]
ax = accel(1);
ay = accel(2);
az = accel(3);

ax = ax + l_h*(gyro(2)^2 + gyro(3)^2); %Fjerner sentripetalaksellerasjonen

if abs(az) < 1e-3
    az = -1e-3;
end

pitch = atan(ay/az);
elevation = atan2(ax, sqrt(ay^2+az^2));

eulerangles = [pitch elevation];
